simulink model "backup2export_ros2_template"  (R2024b)
settings: Solver=ode45  StartTime=0.0  StopTime=inf  MaxStep=0.1  RelTol=1e-3  EnableMultiTasking=on
PreLoadFcn:
  | % load parameters of the default quadrotor
  | disp('Quadrotor parameters loaded by PreLoadFcn')
  | mdl_quadrotor
undefined symbols (not defined in the file or in its folder): angular, linear, rot2
libraries: ros2lib x3, simulink_extras x3
settings Model: Creator=corkep  LastModifiedBy=student
settings SolverCC: AlgebraicLoopSolver=TrustRegion
settings DataIOCC: LimitDataPoints=on  ReturnWorkspaceOutputs=off
settings OptimizationCC: ReuseModelBlockBuffer=off  ExpressionDepthLimit=2147483647  LifeSpan=inf
settings DebuggingCC: UnderspecifiedInitializationDetection=Classic  MergeDetectMultiDrivingBlocksExec=none  SolverPrmCheckMsg=warning  UnconnectedInputMsg=warning  UnconnectedOutputMsg=warning  UnconnectedLineMsg=warning  AllowSymbolicDim=off  StateNameClashWarn=warning  SFUnexpectedBacktrackingDiag=warning  SFNoUnconditionalDefaultTransitionDiag=warning  SFExecutionAtInitializationDiag=none  ArithmeticOperatorsInVariantConditions=warning
settings HardwareCC: ProdBitPerPointer=32  ProdBitPerSizeT=32  ProdBitPerPtrDiffT=32  ProdLargestAtomicFloat=None  ProdIntDivRoundTo=Undefined  ProdEndianess=Unspecified  ProdWordSize=32  ProdHWDeviceType=32-bit Generic
settings ModelReferenceCC: EnableRefExpFcnMdlSchedulingChecks=on  PropagateSignalLabelsOutOfModel=off
settings SFSimCC: SimUseLocalCustomCode=off  CustomCodeUndefinedFunction=UseInterfaceOnly
settings RTWCC: RTWUseLocalCustomCode=off  GPUComputeCapability=3.5  DLArmComputeVersion=19.05
settings CodeAppCC: StateflowObjectComments=on
settings GRTTargetCC: TargetLangStandard=C89/C90 (ANSI)  CombineOutputUpdateFcns=off  GRTInterface=on
settings ConfigComp: CovMetricSettings=dw  CovSaveCumulativeToWorkspaceVar=on  CovSaveSingleToWorkspaceVar=on  CovExternalEMLEnable=off  CovSFcnEnable=off

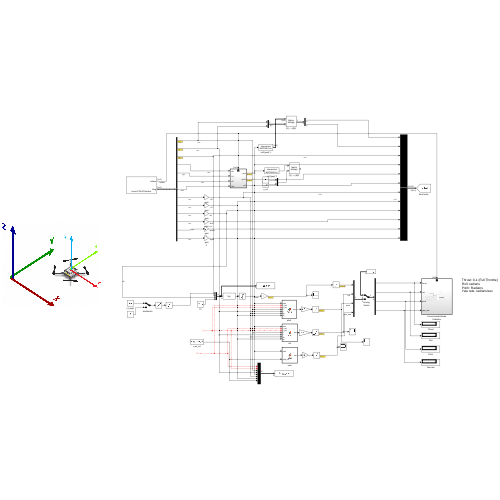
[thumbnail: Simulink's stored preview of the top-level diagram]
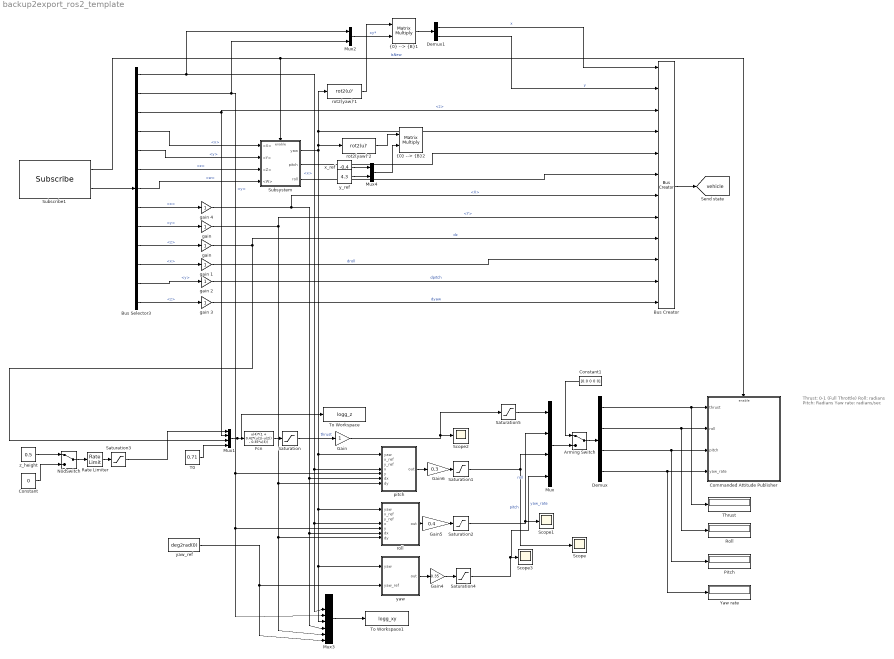
== system backup2export_ros2_template ==
  note: Thrust: 0-1 (Full Throttle)
      | Roll: radians
      | Pitch: Radians
      | Yaw rate: radians/sec
  Arming Switch : ManualSwitch
  Bus Creator : BusCreator  Inputs=12
  Bus Selector3 : BusSelector  OutputSignals=pose.pose.position.x,pose.pose.position.y,pose.pose.position.z,pose.pose.orientation.x,pose.pose.orientation.y,pose.pose.orientation.z,pose.pose.orientation.w,twist.twist.linear.x,twist.twist.linear.y,twist.twist.linear.z,twist.twist.angular.x,twist.twist.angular.y,twist.twist.angular.z
  Commanded Attitude Publisher : Subsystem
  Constant : Constant  Value=0
  Constant1 : Constant  Value=[0.0 0 0 0]
  Demux : Demux
  Demux1 : Demux  Outputs=2
  Fcn : Fcn  Expr=u(4)*(1 + 0.42*(u(1)-u(2)) - 0.35*u(3))
  Gain : Gain
  Gain4 : Gain  Gain=0.35
  Gain5 : Gain  Gain=0.4
  Gain6 : Gain  Gain=0.3
  Mux : Mux
  Mux1 : Mux
  Mux2 : Mux  Inputs=2
  Mux3 : Mux  Inputs=8
  Mux4 : Mux  Inputs=2
  NödSwitch : ManualSwitch
  Pitch : Display
  Rate Limiter : RateLimiter  RisingSlewLimit=0.2  FallingSlewLimit=-0.2  SampleTimeMode=inherited
  Roll : Display
  Saturation : Saturate  UpperLimit=6  LowerLimit=0
  Saturation1 : Saturate  UpperLimit=1  LowerLimit=-1
  Saturation2 : Saturate  UpperLimit=1  LowerLimit=-1
  Saturation3 : Saturate  UpperLimit=1.8  LowerLimit=0
  Saturation4 : Saturate  UpperLimit=1  LowerLimit=-1
  Saturation5 : Saturate  UpperLimit=1  LowerLimit=0
  Scope{,1..3} (4 alike) : Scope
  Subscribe1 : ros2lib/Subscribe  topicSource=Select from ROS network  topic=/vicon/CF6/CF6/odom  messageType=nav_msgs/Odometry  sampleTime=-1  QOSHistory=Keep last  QOSDepth=1  QOSReliability=Reliable  QOSDurability=Volatile  QOSDeadline=Inf  QOSLifespan=Inf  QOSLiveliness=Automatic  QOSLeaseDuration=Inf  QOSAvoidROSNamespaceConventions=off
  Subsystem : Subsystem
  T0 : Constant  Value=0.71
  Thrust : Display
  To Workspace : ToWorkspace  VariableName=logg_z  SaveFormat=Timeseries  SampleTime=-1
  To Workspace1 : ToWorkspace  VariableName=logg_xy  SaveFormat=Timeseries  SampleTime=-1
  Yaw rate : Display
  gain : Gain
  gain {,1..4} (5 alike) : Gain
  pitch : MATLAB Function  TreatAsAtomicUnit=on
  roll : MATLAB Function  TreatAsAtomicUnit=on
  rot2(yaw)'1 : MATLABFcn  MATLABFcn=rot2(u)'  OutputDimensions=[2 2]  Output1D=off
  rot2(yaw)'2 : MATLABFcn  MATLABFcn=rot2(u)'  OutputDimensions=[2 2]  Output1D=off
  x_ref : Constant  Value=-0.4
  y_ref : Constant  Value=4.3
  yaw : MATLAB Function  TreatAsAtomicUnit=on
  yaw_ref : Constant  Value=deg2rad(0)
  z_height : Constant  Value=0.5
  "{0} --> {B}1" : Product  Multiplication=Matrix(*)  RndMeth=Zero
  "{0} --> {B}2" : Product  Multiplication=Matrix(*)  RndMeth=Zero
  tag scope: vehicle=global
  wires:
  Bus Selector3/11 -> gain 1/1  "<x>"
  Bus Selector3/13 -> gain 3/1  "<z>"
  Bus Selector3/10 -> "gain "/1  "<z>"
  Bus Selector3/9 -> gain/1  "<y>"
  Bus Selector3/8 -> gain 4/1  "<x>"
  Bus Creator/1 -> [vehicle]
  Bus Selector3/12 -> gain 2/1  "<y>"
  Subscribe1/2 -> Bus Selector3/1
  Mux2/1 -> "{0} --> {B}1"/2  "xy*"
  "{0} --> {B}1"/1 -> Demux1/1
  Demux1/1 -> Bus Creator/1  "x"
  Demux1/2 -> Bus Creator/2  "y"
  rot2(yaw)'1/1 -> "{0} --> {B}1"/1
  gain 1/1 -> Bus Creator/10  "droll"
  gain 2/1 -> Bus Creator/11  "dpitch"
  gain 3/1 -> Bus Creator/12  "dyaw"
  Bus Selector3/4 -> Subsystem/1(<X>)  "<x>"
  Bus Selector3/5 -> Subsystem/2(<Y>)  "<y>"
  Bus Selector3/6 -> Subsystem/3(<Z>)  "<z>"
  Bus Selector3/7 -> Subsystem/4(<W>)  "<w>"
  Subsystem/2(pitch) -> Bus Creator/5
  Subsystem/3(roll) -> Bus Creator/6
  Subscribe1/1 -> Subsystem/Enable, Commanded Attitude Publisher/Enable  "IsNew"
  Demux/1 -> Thrust/1, Commanded Attitude Publisher/1(thrust)
  Demux/2 -> Roll/1, Commanded Attitude Publisher/2(roll)
  Demux/3 -> Pitch/1, Commanded Attitude Publisher/3(pitch)
  Demux/4 -> Yaw rate/1, Commanded Attitude Publisher/4(yaw_rate)
  Constant1/1 -> Arming Switch/1
  Arming Switch/1 -> Demux/1
  Mux/1 -> Arming Switch/2
  Saturation2/1 -> Mux/2, Scope1/1  "roll"
  Saturation1/1 -> Scope/1, Mux/3  "pitch"
  Saturation4/1 -> Mux/4, Scope3/1  "yaw_rate"
  Mux1/1 -> To Workspace/1, Fcn/1
  Bus Selector3/3 -> Mux1/2, Bus Creator/3  "<z>"
  Rate Limiter/1 -> Saturation3/1
  yaw_ref/1 -> yaw/2(yaw_ref), Mux3/8
  gain/1 -> Bus Creator/8, pitch/7(dy), roll/7(dy), Mux3/7  "<Y>"
  ? -> pitch/2(x_ref), roll/2(x_ref), Mux3/1
  "gain "/1 -> Mux1/3, Bus Creator/9  "dz"
  T0/1 -> Mux1/4
  z_height/1 -> NödSwitch/1
  Mux3/1 -> To Workspace1/1
  NödSwitch/1 -> Rate Limiter/1
  Constant/1 -> NödSwitch/2
  Bus Selector3/2 -> pitch/5(y), roll/5(y), Mux3/4, Mux2/2  "<y>"
  Saturation3/1 -> Mux1/1
  Bus Selector3/1 -> pitch/4(x), roll/4(x), Mux3/3, Mux2/1  "<x>"
  yaw/1(out) -> Gain4/1
  Fcn/1 -> Saturation/1
  ? -> pitch/3(y_ref), roll/3(y_ref), Mux3/2
  gain 4/1 -> Bus Creator/7, pitch/6(dx), roll/6(dx), Mux3/6  "<X>"
  Gain4/1 -> Saturation4/1
  Gain5/1 -> Saturation2/1
  roll/1(out) -> Gain5/1
  pitch/1(out) -> Gain6/1
  Gain6/1 -> Saturation1/1
  Gain/1 -> Saturation5/1, Scope2/1
  Saturation/1 -> Gain/1  "thrust"
  Saturation5/1 -> Mux/1
  Subsystem/1(yaw) -> pitch/1(yaw), roll/1(yaw), yaw/1(yaw), Mux3/5, rot2(yaw)'2/1, rot2(yaw)'1/1, Bus Creator/4
  rot2(yaw)'2/1 -> "{0} --> {B}2"/1
  y_ref/1 -> Mux4/2
  x_ref/1 -> Mux4/1
  Mux4/1 -> "{0} --> {B}2"/2

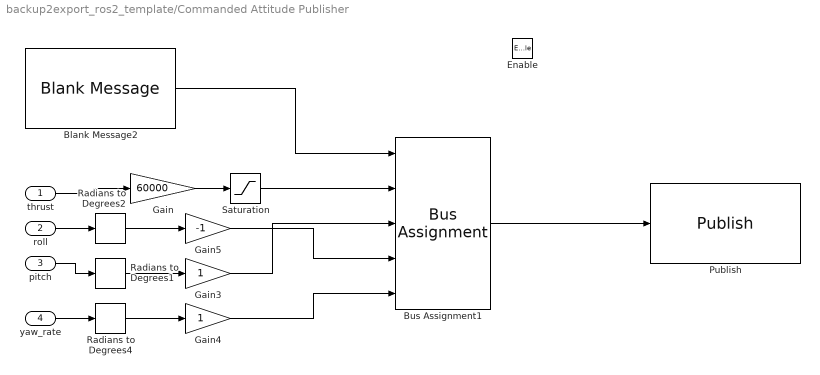
== system backup2export_ros2_template/Commanded Attitude Publisher ==
  thrust : Inport
  roll : Inport  Port=2
  pitch : Inport  Port=3
  yaw_rate : Inport  Port=4
  Enable : EnablePort
  Blank Message2 : ros2lib/Blank Message  messageClass=Message  entityType=geometry_msgs/Twist  messageType=geometry_msgs/Twist  SampleTime=1/30
  Bus Assignment1 : BusAssignment  DialogController=Simulink.DDGSource_BusAssignment  AssignedSignals=linear.z,linear.x,linear.y,angular.z
  Gain : Gain  Gain=60000
  Gain3 : Gain
  Gain4 : Gain
  Gain5 : Gain  Gain=-1
  Publish : ros2lib/Publish  topicSource=Select from ROS network  topic=/cf231/cmd_vel_legacy  messageType=geometry_msgs/Twist  QOSHistory=Keep last  QOSDepth=1  QOSReliability=Reliable  QOSDurability=Volatile  QOSDeadline=Inf  QOSLifespan=Inf  QOSLiveliness=Automatic  QOSLeaseDuration=Inf  QOSAvoidROSNamespaceConventions=off
  Radians to Degrees1 : simulink_extras/Transformations/Radians to Degrees
  Radians to Degrees2 : simulink_extras/Transformations/Radians to Degrees
  Radians to Degrees4 : simulink_extras/Transformations/Radians to Degrees
  Saturation : Saturate  UpperLimit=60000  LowerLimit=0
  wires:
  Bus Assignment1/1 -> Publish/1
  Blank Message2/1 -> Bus Assignment1/1
  thrust/1 -> Gain/1
  Gain/1 -> Saturation/1
  Saturation/1 -> Bus Assignment1/2
  Gain5/1 -> Bus Assignment1/4
  Radians to Degrees2/1 -> Gain5/1
  Radians to Degrees1/1 -> Gain3/1
  Radians to Degrees4/1 -> Gain4/1
  roll/1 -> Radians to Degrees2/1
  pitch/1 -> Radians to Degrees1/1
  Gain3/1 -> Bus Assignment1/3
  yaw_rate/1 -> Radians to Degrees4/1
  Gain4/1 -> Bus Assignment1/5

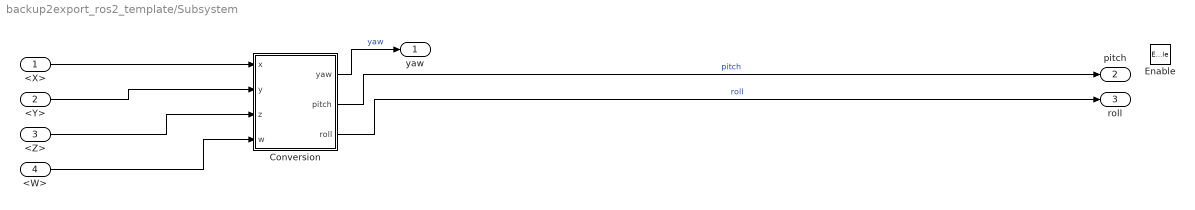
== system backup2export_ros2_template/Subsystem ==
  <X> : Inport
  <Y> : Inport  Port=2
  <Z> : Inport  Port=3
  <W> : Inport  Port=4
  Enable : EnablePort
  Conversion : MATLAB Function  TreatAsAtomicUnit=on
  yaw : Outport
  pitch : Outport  Port=2
  roll : Outport  Port=3
  wires:
  Conversion/1(yaw) -> yaw/1  "yaw"
  <X>/1 -> Conversion/1(x)
  Conversion/2(pitch) -> pitch/1  "pitch"
  <W>/1 -> Conversion/4(w)
  <Y>/1 -> Conversion/2(y)
  Conversion/3(roll) -> roll/1  "roll"
  <Z>/1 -> Conversion/3(z)

== matlab function backup2export_ros2_template/Subsystem/Conversion ==
  data: yaw output; x input; y input; z input; w input; pitch output; roll output
function [yaw,pitch,roll]  = quat2eul(x,y,z,w)
%#codegen

% Convert the quaternion to a yaw angle (zyx euler angle)
eul = quat2eul([w,x,y,z]);
yaw = eul(1);
roll = eul(3);
pitch = eul(2);

end

== matlab function backup2export_ros2_template/pitch ==
  data: yaw input; out output; x_ref input; y_ref input; x input; y input; dx input; dy input
function out = pitch(yaw, x_ref, y_ref, x, y, dx, dy)
% u(1) x_ref
% u(2) y_ref
% u(3) x
% u(4) y
% u(5) yaw
% u(6) dx
% u(7) dy
out= cos(yaw)*(x_ref-x) - dx + sin(yaw)*(y_ref-y) - dy;

== matlab function backup2export_ros2_template/roll ==
  data: yaw input; out output; x_ref input; y_ref input; x input; y input; dx input; dy input
function out = roll(yaw, x_ref, y_ref, x, y, dx, dy)
% u(1) x_ref
% u(2) y_ref
% u(3) x
% u(4) y
% u(5) yaw
% u(6) dx
% u(7) dy
out = -( -sin(yaw)*(x_ref-x) - dx + cos(yaw)*(y_ref-y)  - dy);

== matlab function backup2export_ros2_template/yaw ==
  data: yaw input; out output; yaw_ref input
function out = yaw(yaw, yaw_ref)

out = atan2(sin(yaw_ref-yaw), cos(yaw_ref-yaw));
